simulink model "robust_joint_space_control"  (R2025b)
settings: Solver=ode4  StartTime=0.0  StopTime=120  RelTol=1e-3
undefined symbols (not defined in the file): D, Kd_c, Kp_c, ml, Q, q0, rho_vers, Tc
settings Model: Creator=Valentina Giannotti  LastModifiedBy=giaco
settings OptimizationCC: ReuseModelBlockBuffer=off
settings RTWCC: GPUComputeCapability=3.5

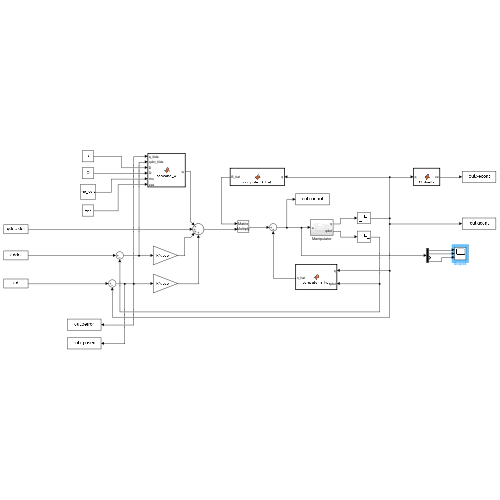
[thumbnail: Simulink's stored preview of the top-level diagram]
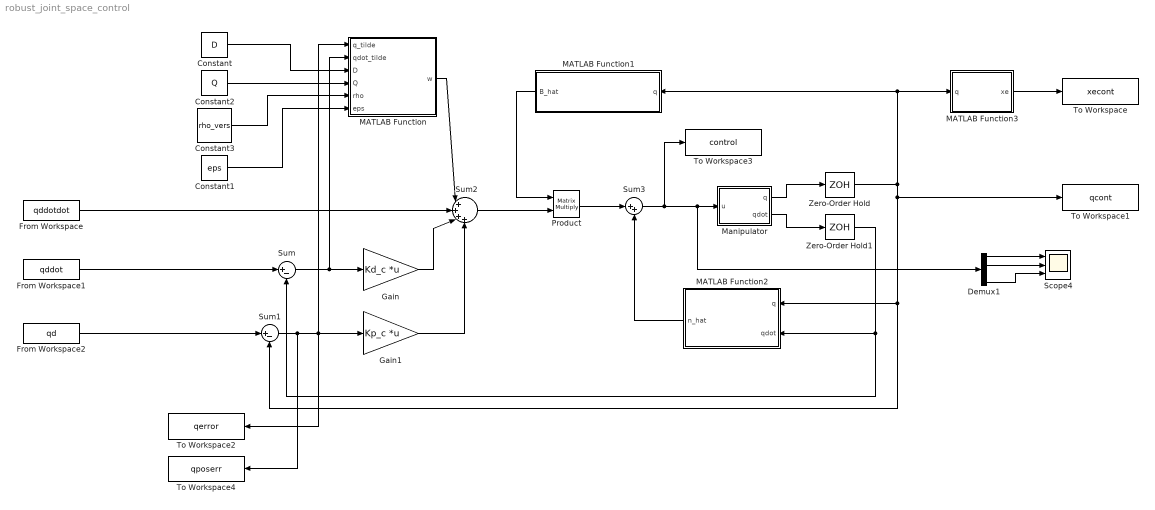
== system robust_joint_space_control ==
  Constant : Constant  Value=D
  Constant1 : Constant  Value=eps
  Constant2 : Constant  Value=Q
  Constant3 : Constant  Value=rho_vers
  Demux1 : Demux
  From Workspace : FromWorkspace  VariableName=qddotdot  SampleTime=Tc
  From Workspace1 : FromWorkspace  VariableName=qddot  SampleTime=Tc
  From Workspace2 : FromWorkspace  VariableName=qd  SampleTime=Tc
  Gain : Gain  Gain=Kd_c  Multiplication=Matrix(K*u) (u vector)
  Gain1 : Gain  Gain=Kp_c  Multiplication=Matrix(K*u) (u vector)
  MATLAB Function : MATLAB Function  TreatAsAtomicUnit=on
  MATLAB Function1 : MATLAB Function  TreatAsAtomicUnit=on
  MATLAB Function2 : MATLAB Function  TreatAsAtomicUnit=on
  MATLAB Function3 : MATLAB Function  TreatAsAtomicUnit=on
  Manipulator : Subsystem
  Product : Product  Multiplication=Matrix(*)
  Scope4 : Scope  NumInputPorts=3
      settings: ActiveDisplayYMinimum=-7.07668  ActiveDisplayYMaximum=5.24775  DataLoggingVariableName=ScopeData4
  Sum : Sum  Inputs=|+-
  Sum1 : Sum  Inputs=|+-
  Sum2 : Sum  Inputs=|++++
  Sum3 : Sum  Inputs=|++
  To Workspace : ToWorkspace  VariableName=xecont  SaveFormat=Structure With Time  SampleTime=-1
  To Workspace1 : ToWorkspace  VariableName=qcont  SaveFormat=Structure With Time  SampleTime=-1
  To Workspace2 : ToWorkspace  VariableName=qerror  SaveFormat=Structure With Time  SampleTime=0.001
  To Workspace3 : ToWorkspace  VariableName=control  SaveFormat=Structure With Time  SampleTime=-1
  To Workspace4 : ToWorkspace  VariableName=qposerr  SaveFormat=Structure With Time  SampleTime=0.001
  Zero-Order Hold : ZeroOrderHold  SampleTime=Tc
  Zero-Order Hold1 : ZeroOrderHold  SampleTime=Tc
  wires:
  Gain/1 -> Sum2/3
  From Workspace/1 -> Sum2/2
  Manipulator/1(q) -> Zero-Order Hold/1
  Zero-Order Hold1/1 -> Sum/2, MATLAB Function2/2(qdot)
  From Workspace1/1 -> Sum/1
  MATLAB Function3/1(xe) -> To Workspace/1
  Constant1/1 -> MATLAB Function/6(eps)
  MATLAB Function/1(w) -> Sum2/1
  MATLAB Function1/1(B_hat) -> Product/1
  Sum2/1 -> Product/2
  Manipulator/2(qdot) -> Zero-Order Hold1/1
  MATLAB Function2/1(n_hat) -> Sum3/2
  Zero-Order Hold/1 -> MATLAB Function2/1(q), Sum1/2, To Workspace1/1, MATLAB Function3/1(q), MATLAB Function1/1(q)
  Gain1/1 -> Sum2/4
  Constant/1 -> MATLAB Function/3(D)
  Sum3/1 -> To Workspace3/1, Demux1/1, Manipulator/1(u)
  Constant3/1 -> MATLAB Function/5(rho)
  Sum1/1 -> To Workspace4/1, MATLAB Function/1(q_tilde), Gain1/1, To Workspace2/1
  Product/1 -> Sum3/1
  From Workspace2/1 -> Sum1/1
  Constant2/1 -> MATLAB Function/4(Q)
  Sum/1 -> MATLAB Function/2(qdot_tilde), Gain/1
  Demux1/1 -> Scope4/1
  Demux1/2 -> Scope4/2
  Demux1/4 -> Scope4/3

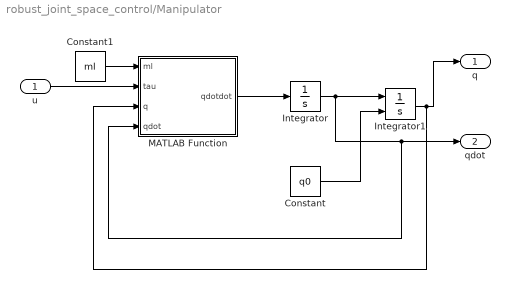
== system robust_joint_space_control/Manipulator ==
  u : Inport
  Constant : Constant  Value=q0
  Constant1 : Constant  Value=ml
  Integrator : Integrator  InitialCondition=[0 0 0 0]'
  Integrator1 : Integrator  InitialConditionSource=external
  MATLAB Function : MATLAB Function  TreatAsAtomicUnit=on
  q : Outport
  qdot : Outport  Port=2
  wires:
  u/1 -> MATLAB Function/2(tau)
  MATLAB Function/1(qdotdot) -> Integrator/1
  Integrator/1 -> MATLAB Function/4(qdot), qdot/1, Integrator1/1
  Constant/1 -> Integrator1/2
  Integrator1/1 -> MATLAB Function/3(q), q/1
  Constant1/1 -> MATLAB Function/1(ml)

== matlab function robust_joint_space_control/MATLAB Function ==
  data: q_tilde input; w output; qdot_tilde input; D input; Q input; rho input; eps input
function w = compute_w(q_tilde,qdot_tilde,D,Q,rho,eps)
% Use a linear correction near zero to reduce chattering.

xi = [q_tilde;qdot_tilde];
z = D'*Q*xi;

if norm(z) >= eps
    w = rho*(z/norm(z));
else
    w = rho*(z/eps);
end

end

== matlab function robust_joint_space_control/MATLAB Function1 ==
  data: q input; B_hat output
function B_hat = compute_B_hat(q)
% Joint-space inertia with the nominal load.

a1=0.5;
a2=0.5;
l1=0.25;
l2=0.25;
ml1=20;
ml2=20;
ml3=10;
Il1=4;
Il2=4;
Il4=1;
kr1=1;
kr2=1;
kr3=50;
kr4=20;
Im1=0.01;
Im2=0.01;
Im3=0.005;
Im4=0.001;

mhe=0; % Payload mass parameter [kg]

% Link and rotor Jacobians used to assemble the inertia matrix.
Jpl1=[-l1*sin(q(1)) 0 0 0;
    l1*cos(q(1)) 0 0 0;
    0 0 0 0];

Jpl2=[-a1*sin(q(1))-l2*sin(q(1)+q(2)),-l2*sin(q(1)+q(2)),0,0;
    a1*cos(q(1))+l2*cos(q(1)+q(2)),l2*cos(q(1)+q(2)),0,0;
    0,0,0,0];

Jpl4=[-a1*sin(q(1))-a2*sin(q(1)+q(2)),-a2*sin(q(1)+q(2)),0,0;
    a1*cos(q(1))+a2*cos(q(1)+q(2)),a2*cos(q(1)+q(2)),0,0;
    0,0,1,0];

Jol1=[zeros(2,4);
    1 0 0 0];

Jol2=[zeros(2,4);
    1 1 0 0];

Jol4=[zeros(2,4);
    1 1 0 1];

Jom1=[zeros(2,4);
    kr1 0 0 0];

Jom2=[zeros(2,4);
    1 kr2 0 0];

Jom3=[zeros(2,4);
    1 1 kr3 0];

Jom4=[zeros(2,4);
    1 1 0 kr4];

B = ml1*(Jpl1'*Jpl1)+Jol1'*Il1*Jol1+Jom1'*Im1*Jom1...
    +ml2*(Jpl2'*Jpl2)+Jol2'*Il2*Jol2+Jom2'*Im2*Jom2...
    +Jom3'*Im3*Jom3...
    +(mhe+ml3)*(Jpl4'*Jpl4)+Jol4'*Il4*Jol4+Jom4'*Im4*Jom4;

B_hat = diag([B(1,1), B(2,2), B(3,3), B(4,4)]);

end

== matlab function robust_joint_space_control/MATLAB Function2 ==
  data: q input; n_hat output; qdot input
function n_hat = compute_n_hat(q,qdot)
% The nominal model compensates friction and gravity.

a1=0.5;
a2=0.5;
l1=0.25;
l2=0.25;
ml1=20;
ml2=20;
ml3=10;
Il1=4;
Il2=4;
Il4=1;
kr1=1;
kr2=1;
kr3=50;
kr4=20;
Im1=0.01;
Im2=0.01;
Im3=0.005;
Im4=0.001;
Fm1=0.00005;
Fm2=0.00005;
Fm3=0.01;
Fm4=0.005;

g=[0 0 9.81*(ml3) 0]';

Fv=diag([kr1^2*Fm1,kr2^2*Fm2,kr3^2*Fm3,kr4^2*Fm4]);

n_hat = Fv*qdot+g;

== matlab function robust_joint_space_control/Manipulator/MATLAB Function ==
  data: ml input; qdotdot output; tau input; q input; qdot input
function qdotdot= dinamica_diretta(ml,tau,q,qdot)
% Plant dynamics: subtract Coriolis, friction, and gravity before solving for acceleration.

a1=0.5;
a2=0.5;
l1=0.25;
l2=0.25;
ml1=20;
ml2=20;
ml3=10;
Il1=4;
Il2=4;
Il4=1;
kr1=1;
kr2=1;
kr3=50;
kr4=20;
Im1=0.01;
Im2=0.01;
Im3=0.005;
Im4=0.001;

Fm1=0.00005;
Fm2=0.00005;
Fm3=0.01;
Fm4=0.005;

% Link and rotor Jacobians used to assemble the inertia matrix.
Jpl1=[-l1*sin(q(1)) 0 0 0;
    l1*cos(q(1)) 0 0 0;
    0 0 0 0];

Jpl2=[-a1*sin(q(1))-l2*sin(q(1)+q(2)),-l2*sin(q(1)+q(2)),0,0;
    a1*cos(q(1))+l2*cos(q(1)+q(2)),l2*cos(q(1)+q(2)),0,0;
    0,0,0,0];

Jpl4=[-a1*sin(q(1))-a2*sin(q(1)+q(2)),-a2*sin(q(1)+q(2)),0,0;
    a1*cos(q(1))+a2*cos(q(1)+q(2)),a2*cos(q(1)+q(2)),0,0;
    0,0,1,0];

Jol1=[zeros(2,4);
    1 0 0 0];

Jol2=[zeros(2,4);
    1 1 0 0];

Jol4=[zeros(2,4);
    1 1 0 1];

Jom1=[zeros(2,4);
    kr1 0 0 0];

Jom2=[zeros(2,4);
    1 kr2 0 0];

Jom3=[zeros(2,4);
    1 1 kr3 0];

Jom4=[zeros(2,4);
    1 1 0 kr4];

B=ml1*(Jpl1'*Jpl1)...
+Jol1'*Il1*Jol1...
+Jom1'*Im1*Jom1...
+ml2*(Jpl2'*Jpl2)...
+Jol2'*Il2*Jol2...
+Jom2'*Im2*Jom2...
+Jom3'*Im3*Jom3...
+(ml+ml3)*(Jpl4'*Jpl4)...
+Jol4'*Il4*Jol4...
+Jom4'*Im4*Jom4;

c=zeros(4,4,4);

Jpl1dq1=[-l1*cos(q(1)) 0 0 0;
    -l1*sin(q(1)) 0 0 0;
    0 0 0 0];

Jpl1dq2=zeros(3,4);

Jpl2dq1=[-a1*cos(q(1))-l2*cos(q(1)+q(2)),-l2*cos(q(1)+q(2)),0,0;
    -a1*sin(q(1))-l2*sin(q(1)+q(2)),-l2*sin(q(1)+q(2)),0,0;
    0,0,0,0];

Jpl2dq2=[-l2*cos(q(1)+q(2)),-l2*cos(q(1)+q(2)),0,0;
    -l2*sin(q(1)+q(2)),-l2*sin(q(1)+q(2)),0,0;
    0,0,0,0];

Jpl4dq1=[-a1*cos(q(1))-a2*cos(q(1)+q(2)),-a2*cos(q(1)+q(2)),0,0;
    -a1*sin(q(1))-a2*sin(q(1)+q(2)),-a2*sin(q(1)+q(2)),0,0;
    0,0,0,0];

Jpl4dq2=[-a2*cos(q(1)+q(2)),-a2*cos(q(1)+q(2)),0,0;
    -a2*sin(q(1)+q(2)),-a2*sin(q(1)+q(2)),0,0;
    0,0,0,0];

dBdq1=ml1*(Jpl1dq1'*Jpl1+Jpl1'*Jpl1dq1)+ml2*(Jpl2dq1'*Jpl2+Jpl2'*Jpl2dq1)+ml3*(Jpl4dq1'*Jpl4+Jpl4'*Jpl4dq1);
dBdq2=ml1*(Jpl1dq2'*Jpl1+Jpl1'*Jpl1dq2)+ml2*(Jpl2dq2'*Jpl2+Jpl2'*Jpl2dq2)+ml3*(Jpl4dq2'*Jpl4+Jpl4'*Jpl4dq2);

c(1,1,2)=-ml2*a1*l2*sin(q(2))-ml3*a1*a2*sin(q(2));
c(1,2,2)=c(1,1,2);
c(2,1,1)=-c(1,1,2);

C=zeros(4,4);
    for i=1:4
        for j=1:4
            for k=1:4
                C(i,j)=c(i,j,k)*qdot(k);
            end
        end
    end

g=[0 0 9.81*(ml+ml3) 0]';

Fv=diag([kr1^2*Fm1,kr2^2*Fm2,kr3^2*Fm3,kr4^2*Fm4]);
qdotdot=inv(B)*(tau-C*qdot-Fv*qdot-g);
end

== matlab function robust_joint_space_control/MATLAB Function3 ==
  data: q input; xe output
function xe = C_diretta(q)
% Pose in base coordinates, ordered as [x; y; z; phi].
a1=0.5;
a2=a1;
d0=1;

xe=[a1*cos(q(1))+a2*cos(q(1)+q(2));...
    a1*sin(q(1))+a2*sin(q(1)+q(2));...
    d0+q(3);...
    q(1)+q(2)+q(4)];
end
